simulink model "AFC_FFNN_trainscg_15_15_15_15_15_ctr_Nor_July_15"  (R2021a)
settings: Solver=VariableStepAuto  StartTime=0.0  StopTime=10.0  RelTol=1e-3
libraries: neural x82
(part 2 of 3)

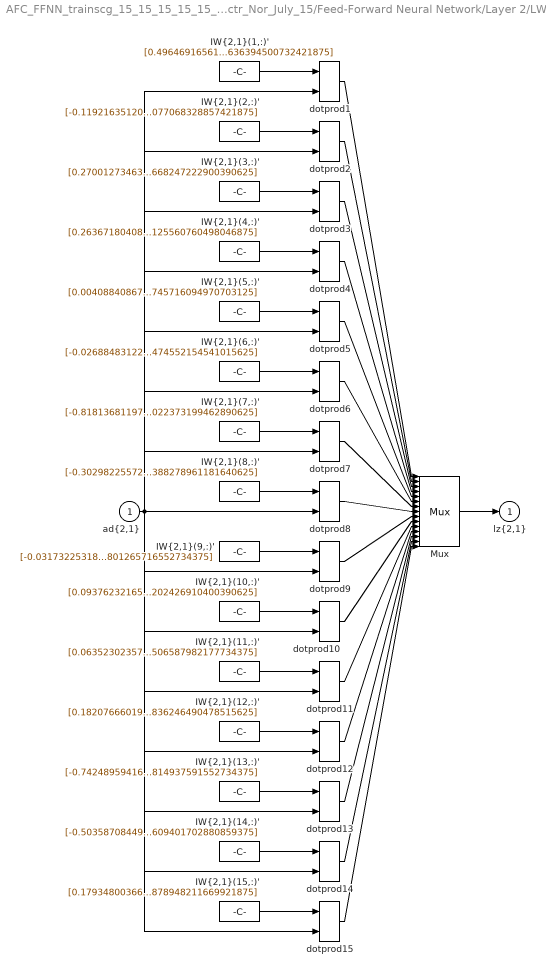
== system AFC_FFNN_trainscg_15_15_15_15_15_ctr_Nor_July_15/Feed-Forward Neural Network/Layer 2/LW{2,1} ==
  "ad{2,1}" : Inport  PortDimensions=15
      mask Display: e = 0.06;c1 = [120 230 180]/255;c2 = ([120 230 180]+0)/(256+128);c3 = ([120 230 180]+128)/(256+128);patch([0 1 1 0],[0 0 1 1],c1);patch([0 1 1 1-e 1-e 0+e],[0 0 1 1-e 0+e 0+e],c2);patch([0 0 1 1-e 0+e 0+e],[0 1 1 1-e 1-e 0+e],c3);plot([0 1 1 0 0],[0 0 1 1 0]);
  "IW{2,1}(1,:)'" : Constant  Value=[0.49646916561011245061507679565693251788616180419921875;0.77996133484927110401940808515064418315887451171875;-0.4843167782638080343105002611991949379444122314453125;0.91967297978227990906674449433921836316585540771484375;0.8707941521523403505256055723293684422969818115234375;0.5037557738819355979131842104834504425525665283203125;-0.7017295301971968601861817660392262041568756103515625;0.309274426520241119131782170370570383965969085693359375;0.90641457105355194290297049519722349941730499267578125;0.10882574325775402901417265866257366724312305450439453125;0.90673057127212108863290040972060523927211761474609375;-0.80524588547048792097626801478327251970767974853515625;0.104579561651616914641493849558173678815364837646484375;-0.386551898471740595919499128285679034888744354248046875;0.4908219201017736121883672240073792636394500732421875]
      mask Display: e = 0.06;c1 = [120 150 230]/255;c2 = ([120 150 230]+0)/383;c3 = ([120 150 230]+128)/383;patch([0 1 1 0],[0 0 1 1],c1);patch([0 1 1 1-e 1-e 0+e],[0 0 1 1-e 0+e 0+e],c2);patch([0 0 1 1-e 0+e 0+e],[0 1 1 1-e 1-e 0+e],c3);plot([0 1 1 0 0],[0 0 1 1 0]);disp('weights');
  "IW{2,1}(10,:)'" : Constant  Value=[0.0937623216569043460566490466590039432048797607421875;0.77106293047639129500936405747779645025730133056640625;0.4586134724193680067827472157659940421581268310546875;-0.7860483088632481685209540955838747322559356689453125;-0.52866293231569916333256742291268892586231231689453125;0.6383602490350686053943718434311449527740478515625;0.342034306689907363629998826581868343055248260498046875;0.212238388955804213598099750015535391867160797119140625;-0.976573937691504578850754114682786166667938232421875;0.64814439757751340920322036254219710826873779296875;-0.88015675771774992686147243148298002779483795166015625;-0.537524641968443628314844318083487451076507568359375;-0.552249744431198674732286235666833817958831787109375;-0.32473785236878993654130454160622321069240570068359375;-0.11032019079443211584390382995479740202426910400390625]
      mask Display: e = 0.06;c1 = [120 150 230]/255;c2 = ([120 150 230]+0)/383;c3 = ([120 150 230]+128)/383;patch([0 1 1 0],[0 0 1 1],c1);patch([0 1 1 1-e 1-e 0+e],[0 0 1 1-e 0+e 0+e],c2);patch([0 0 1 1-e 0+e 0+e],[0 1 1 1-e 1-e 0+e],c3);plot([0 1 1 0 0],[0 0 1 1 0]);disp('weights');
  "IW{2,1}(11,:)'" : Constant  Value=[0.06352302357512840114139862635056488215923309326171875;0.77580634612318088993987430512788705527782440185546875;0.4976683056216459899445681003271602094173431396484375;0.710615284497925880913271612371318042278289794921875;0.0284508200153920677577534803504022420383989810943603515625;-0.4262598504785959363516667508520185947418212890625;0.79535543465944924523824965945095755159854888916015625;-0.50420641521105835636262781918048858642578125;-0.78178862131788517952912798136821947991847991943359375;0.64520731580435242147331109663355164229869842529296875;0.8267663858165315016179874874069355428218841552734375;-0.480465110495678582314127424979233182966709136962890625;0.53645329785536877142959610864636488258838653564453125;0.09182180567506821600165523022951674647629261016845703125;-0.2422337966092920902294594043269171379506587982177734375]
      mask Display: e = 0.06;c1 = [120 150 230]/255;c2 = ([120 150 230]+0)/383;c3 = ([120 150 230]+128)/383;patch([0 1 1 0],[0 0 1 1],c1);patch([0 1 1 1-e 1-e 0+e],[0 0 1 1-e 0+e 0+e],c2);patch([0 0 1 1-e 0+e 0+e],[0 1 1 1-e 1-e 0+e],c3);plot([0 1 1 0 0],[0 0 1 1 0]);disp('weights');
  "IW{2,1}(12,:)'" : Constant  Value=[0.182076660191047789982832227906328625977039337158203125;0.0361498754295182800344576889983727596700191497802734375;0.943422814506380991161904603359289467334747314453125;-0.07051674807384201992821459725746535696089267730712890625;-0.91829558979760783632428911005263216793537139892578125;0.7502905528531134127234736297396011650562286376953125;0.496483911800009891646112691887537948787212371826171875;0.59923945203563711014993486969615332782268524169921875;-0.3292028577878360895425657872692681849002838134765625;-0.13105378107113896390956142568029463291168212890625;0.80434019538809276017587990281754173338413238525390625;0.249007566369504773629017790881334803998470306396484375;-0.89566786392105457448309380197315476834774017333984375;0.9758812474243507839588573915534652769565582275390625;-0.3177526207662977331125375712872482836246490478515625]
      mask Display: e = 0.06;c1 = [120 150 230]/255;c2 = ([120 150 230]+0)/383;c3 = ([120 150 230]+128)/383;patch([0 1 1 0],[0 0 1 1],c1);patch([0 1 1 1-e 1-e 0+e],[0 0 1 1-e 0+e 0+e],c2);patch([0 0 1 1-e 0+e 0+e],[0 1 1 1-e 1-e 0+e],c3);plot([0 1 1 0 0],[0 0 1 1 0]);disp('weights');
  "IW{2,1}(13,:)'" : Constant  Value=[-0.7424895941637081886455007406766526401042938232421875;-0.856648876074442622297056004754267632961273193359375;0.4489983138356112846167889074422419071197509765625;0.0342511534493581404348105934332124888896942138671875;-0.1478990255038865608838705156813375651836395263671875;-0.727415351703474044597896863706409931182861328125;-0.7367400157489829570778283596155233681201934814453125;0.0653226259463746128375305488589219748973846435546875;-0.089870329604618603980270563624799251556396484375;0.0129175888645709502355884978896938264369964599609375;0.8733140785372424108601308034849353134632110595703125;-0.2333190812499730260043406815384514629840850830078125;-0.72095782901882099480417309678159654140472412109375;-0.6008520238705161720105252243229188024997711181640625;-0.9615455944680115774048090315773151814937591552734375]
      mask Display: e = 0.06;c1 = [120 150 230]/255;c2 = ([120 150 230]+0)/383;c3 = ([120 150 230]+128)/383;patch([0 1 1 0],[0 0 1 1],c1);patch([0 1 1 1-e 1-e 0+e],[0 0 1 1-e 0+e 0+e],c2);patch([0 0 1 1-e 0+e 0+e],[0 1 1 1-e 1-e 0+e],c3);plot([0 1 1 0 0],[0 0 1 1 0]);disp('weights');
  "IW{2,1}(14,:)'" : Constant  Value=[-0.50358708449105638038645338383503258228302001953125;0.98956782330111947576511965962708927690982818603515625;-0.2361487675618059167703677303506992757320404052734375;0.007202825434977723484397671427359455265104770660400390625;-0.54195442663654513903992437917622737586498260498046875;0.95067385879104904233827255666255950927734375;-0.492871953524475603369836562706041149795055389404296875;-0.838459952423429744072791436337865889072418212890625;0.7937041538789466610381850841804407536983489990234375;0.59786126522488303169922119195689447224140167236328125;0.40169531108736389324320725791039876639842987060546875;-0.11999535239950331888536538826883770525455474853515625;0.3818939688303688573256522431620396673679351806640625;0.28629620337122674289531687463750131428241729736328125;0.306668631161549354313677895333967171609401702880859375]
      mask Display: e = 0.06;c1 = [120 150 230]/255;c2 = ([120 150 230]+0)/383;c3 = ([120 150 230]+128)/383;patch([0 1 1 0],[0 0 1 1],c1);patch([0 1 1 1-e 1-e 0+e],[0 0 1 1-e 0+e 0+e],c2);patch([0 0 1 1-e 0+e 0+e],[0 1 1 1-e 1-e 0+e],c3);plot([0 1 1 0 0],[0 0 1 1 0]);disp('weights');
  "IW{2,1}(15,:)'" : Constant  Value=[0.1793480036698109625348251938703469932079315185546875;-0.1774866557153116364276002059341408312320709228515625;0.0058018808544819666650482758996076881885528564453125;-0.43136233850821792401575294206850230693817138671875;0.6441880721956698696573084816918708384037017822265625;0.9393437732971190445852016637218184769153594970703125;-0.4988861248860751995692908167256973683834075927734375;0.1004589318309039303045437918626703321933746337890625;-0.874463826702308377747385748079977929592132568359375;0.301052562896285902382942367694340646266937255859375;-0.477452557381994768803679107804782688617706298828125;-0.759402127653759695391499917604960501194000244140625;-0.9407295984391181864481268348754383623600006103515625;-0.7407365473768721120251257161726243793964385986328125;0.8829622103937289079311767636681906878948211669921875]
      mask Display: e = 0.06;c1 = [120 150 230]/255;c2 = ([120 150 230]+0)/383;c3 = ([120 150 230]+128)/383;patch([0 1 1 0],[0 0 1 1],c1);patch([0 1 1 1-e 1-e 0+e],[0 0 1 1-e 0+e 0+e],c2);patch([0 0 1 1-e 0+e 0+e],[0 1 1 1-e 1-e 0+e],c3);plot([0 1 1 0 0],[0 0 1 1 0]);disp('weights');
  "IW{2,1}(2,:)'" : Constant  Value=[-0.11921635120059757839694469794267206452786922454833984375;-0.607546895104995154923699374194256961345672607421875;0.5900632710409168257825740511179901659488677978515625;-0.138270521887720487796968882321380078792572021484375;0.94863459152685891684342323060263879597187042236328125;0.108212254673193175591450199135579168796539306640625;0.6336456199801230315671318749082274734973907470703125;-0.852210835717297499058986431919038295745849609375;0.499621559800357439851126173380180262029170989990234375;0.324437729528092744235578948064357973635196685791015625;-0.450664172986721733860093763723853044211864471435546875;-0.53748757708461780691067133375327102839946746826171875;0.1466756409986354758867577174896723590791225433349609375;0.9207406241604727537009011939517222344875335693359375;0.6230024512652061474682341213338077068328857421875]
      mask Display: e = 0.06;c1 = [120 150 230]/255;c2 = ([120 150 230]+0)/383;c3 = ([120 150 230]+128)/383;patch([0 1 1 0],[0 0 1 1],c1);patch([0 1 1 1-e 1-e 0+e],[0 0 1 1-e 0+e 0+e],c2);patch([0 0 1 1-e 0+e 0+e],[0 1 1 1-e 1-e 0+e],c3);plot([0 1 1 0 0],[0 0 1 1 0]);disp('weights');
  "IW{2,1}(3,:)'" : Constant  Value=[0.2700127346397784844356237954343669116497039794921875;-0.9047528966046705090064961041207425296306610107421875;-0.430330309352361606300974017358385026454925537109375;-0.6030524532782468583036461495794355869293212890625;0.6380385707500888514687176211737096309661865234375;0.54795002035806472662216037861071527004241943359375;0.005250284302730445773477185866795480251312255859375;-0.1241388584709621767387943691574037075042724609375;-0.535917014359012622293221284053288400173187255859375;-0.7535723587361520259264580090530216693878173828125;-0.6954156221470046972399359219707548618316650390625;-0.1377055300142842053645608757506124675273895263671875;0.9674587418212110545567838926217518746852874755859375;-0.366043734123321140572215881547890603542327880859375;0.27252194091142545318007250898517668247222900390625]
      mask Display: e = 0.06;c1 = [120 150 230]/255;c2 = ([120 150 230]+0)/383;c3 = ([120 150 230]+128)/383;patch([0 1 1 0],[0 0 1 1],c1);patch([0 1 1 1-e 1-e 0+e],[0 0 1 1-e 0+e 0+e],c2);patch([0 0 1 1-e 0+e 0+e],[0 1 1 1-e 1-e 0+e],c3);plot([0 1 1 0 0],[0 0 1 1 0]);disp('weights');
  "IW{2,1}(4,:)'" : Constant  Value=[0.263671804087154904028267310422961600124835968017578125;-0.088848657628518290518826461266144178807735443115234375;0.319605914056265039135951155913062393665313720703125;0.43228381383499936418957076966762542724609375;-0.50480747820906402001384094546665437519550323486328125;0.5334080567160881525268223413149826228618621826171875;0.24319585957480349680537301537697203457355499267578125;0.0781634291431403394057042532949708402156829833984375;0.42457360577352798447492432387662120163440704345703125;0.419709979053071668975150032565579749643802642822265625;0.064052803186310125482805233332328498363494873046875;0.1443572233574179353166044847966986708343029022216796875;0.499054679010293267271691775022190995514392852783203125;-0.95638137624631947009135046755545772612094879150390625;0.73648140912501414145907574493321590125560760498046875]
      mask Display: e = 0.06;c1 = [120 150 230]/255;c2 = ([120 150 230]+0)/383;c3 = ([120 150 230]+128)/383;patch([0 1 1 0],[0 0 1 1],c1);patch([0 1 1 1-e 1-e 0+e],[0 0 1 1-e 0+e 0+e],c2);patch([0 0 1 1-e 0+e 0+e],[0 1 1 1-e 1-e 0+e],c3);plot([0 1 1 0 0],[0 0 1 1 0]);disp('weights');
  "IW{2,1}(5,:)'" : Constant  Value=[0.00408840867784126572870295746042756945826113224029541015625;0.09388048935012498208418918466122704558074474334716796875;-0.991924688688980982220755322487093508243560791015625;-0.8552316983080421319840525029576383531093597412109375;-0.1911860906079498878540334771969355642795562744140625;0.366618630720363825048480066470801830291748046875;0.7860653630786631484994586571701802313327789306640625;0.37038892020122304860052508956869132816791534423828125;-0.8905075787511116391925725110922940075397491455078125;-0.50182237106303106966009863754152320325374603271484375;0.7785018803667196340967393553000874817371368408203125;0.7206772319558594208643853562534786760807037353515625;-0.07958944169128155665671187080079107545316219329833984375;0.8513328940182223192323363036848604679107666015625;-0.9719425482959789253101234862697310745716094970703125]
      mask Display: e = 0.06;c1 = [120 150 230]/255;c2 = ([120 150 230]+0)/383;c3 = ([120 150 230]+128)/383;patch([0 1 1 0],[0 0 1 1],c1);patch([0 1 1 1-e 1-e 0+e],[0 0 1 1-e 0+e 0+e],c2);patch([0 0 1 1-e 0+e 0+e],[0 1 1 1-e 1-e 0+e],c3);plot([0 1 1 0 0],[0 0 1 1 0]);disp('weights');
  "IW{2,1}(6,:)'" : Constant  Value=[-0.0268848312263405588018461145338733331300318241119384765625;0.9246644738401335050781426616595126688480377197265625;-0.3050290799498984739557272405363619327545166015625;0.38414616541861434928506469077547080814838409423828125;0.034637294652763044033871864257889683358371257781982421875;0.625021902709288923460917430929839611053466796875;0.5043207504740092605999279840034432709217071533203125;0.1342838675116662938702205565277836285531520843505859375;-0.271313482373797321134389903818373568356037139892578125;0.4706688023118104080566581615130417048931121826171875;0.192185046668555903348618585368967615067958831787109375;0.903737226583765984599949661060236394405364990234375;-0.191130177012016011506290169563726522028446197509765625;-0.45184982043038257604194996019941754639148712158203125;-0.45605259254523444756301842062384821474552154541015625]
      mask Display: e = 0.06;c1 = [120 150 230]/255;c2 = ([120 150 230]+0)/383;c3 = ([120 150 230]+128)/383;patch([0 1 1 0],[0 0 1 1],c1);patch([0 1 1 1-e 1-e 0+e],[0 0 1 1-e 0+e 0+e],c2);patch([0 0 1 1-e 0+e 0+e],[0 1 1 1-e 1-e 0+e],c3);plot([0 1 1 0 0],[0 0 1 1 0]);disp('weights');
  "IW{2,1}(7,:)'" : Constant  Value=[-0.8181368119719962805902468971908092498779296875;-0.2417652257721003561385941793560050427913665771484375;0.77475446764487099216012211400084197521209716796875;-0.8479136503999418206234395256615243852138519287109375;-0.1962586542624291663372559924027882516384124755859375;-0.8289192649386392108823429225594736635684967041015625;-0.5728176091748220510879718858632259070873260498046875;-0.509054777740965302967879324569366872310638427734375;0.595048053803708398845628835260868072509765625;-0.0668896360863564520826685111387632787227630615234375;-0.723707884416889601908451368217356503009796142578125;-0.110236535200048280103146680630743503570556640625;-0.0815360751524158988701174166635610163211822509765625;-0.7837666978321446986655018918099813163280487060546875;0.676385977534560201007707291864790022373199462890625]
      mask Display: e = 0.06;c1 = [120 150 230]/255;c2 = ([120 150 230]+0)/383;c3 = ([120 150 230]+128)/383;patch([0 1 1 0],[0 0 1 1],c1);patch([0 1 1 1-e 1-e 0+e],[0 0 1 1-e 0+e 0+e],c2);patch([0 0 1 1-e 0+e 0+e],[0 1 1 1-e 1-e 0+e],c3);plot([0 1 1 0 0],[0 0 1 1 0]);disp('weights');
  "IW{2,1}(8,:)'" : Constant  Value=[-0.302982255725591453909828487667255103588104248046875;0.8981066832894628593209063183167017996311187744140625;0.7377501160157395876382224741973914206027984619140625;-0.51436050278973510785363032482564449310302734375;-0.974697580153902176647306987433694303035736083984375;0.7051429342498158892027504407451488077640533447265625;0.4605206164095310139572347907233051955699920654296875;-0.373094973925372386247545364312827587127685546875;0.162026455868859553532956851995550096035003662109375;0.0954318321609530784144226345233619213104248046875;-0.53521495323957424261607229709625244140625;-0.0899306950871696653138087640400044620037078857421875;-0.41688631732145697839087006286717951297760009765625;-0.75233462966951680783722622436471283435821533203125;-0.5567396324852271760619260021485388278961181640625]
      mask Display: e = 0.06;c1 = [120 150 230]/255;c2 = ([120 150 230]+0)/383;c3 = ([120 150 230]+128)/383;patch([0 1 1 0],[0 0 1 1],c1);patch([0 1 1 1-e 1-e 0+e],[0 0 1 1-e 0+e 0+e],c2);patch([0 0 1 1-e 0+e 0+e],[0 1 1 1-e 1-e 0+e],c3);plot([0 1 1 0 0],[0 0 1 1 0]);disp('weights');
  "IW{2,1}(9,:)'" : Constant  Value=[-0.03173225318246419845991113106720149517059326171875;-0.552686190513204333996100103831849992275238037109375;0.540447992482629313570896556484512984752655029296875;0.50729806833549417888207244686782360076904296875;-0.1229728520261097468591060533071868121623992919921875;0.612215314341371996675889022299088537693023681640625;-0.6820196650305467844788154252455569803714752197265625;0.7640746318530091674148252423037774860858917236328125;0.9475084056062905712991550899459980428218841552734375;0.406609182665139012868849022197537124156951904296875;-0.231903100212810020508413799689151346683502197265625;-0.83148171255660230372086516581475734710693359375;-0.5010392717716840582653503588517196476459503173828125;-0.443925165630052021015217178501188755035400390625;0.3313515085669587190153606570675037801265716552734375]
      mask Display: e = 0.06;c1 = [120 150 230]/255;c2 = ([120 150 230]+0)/383;c3 = ([120 150 230]+128)/383;patch([0 1 1 0],[0 0 1 1],c1);patch([0 1 1 1-e 1-e 0+e],[0 0 1 1-e 0+e 0+e],c2);patch([0 0 1 1-e 0+e 0+e],[0 1 1 1-e 1-e 0+e],c3);plot([0 1 1 0 0],[0 0 1 1 0]);disp('weights');
  Mux : Mux  Inputs=15
      mask Display: e = 0.06;c1 = [120 150 230]/255;c2 = ([120 150 230]+0)/383;c3 = ([120 150 230]+128)/383;patch([0 1 1 0],[0 0 1 1],c1);patch([0 1 1 1-e 1-e 0+e],[0 0 1 1-e 0+e 0+e],c2);patch([0 0 1 1-e 0+e 0+e],[0 1 1 1-e 1-e 0+e],c3);plot([0 1 1 0 0],[0 0 1 1 0]);disp('Mux');
  dotprod{1..15} (15 alike) : neural/Weight Functions/dotprod
  "lz{2,1}" : Outport
      mask Display: e = 0.06;c1 = [120 230 180]/255;c2 = ([120 230 180]+0)/(256+128);c3 = ([120 230 180]+128)/(256+128);patch([0 1 1 0],[0 0 1 1],c1);patch([0 1 1 1-e 1-e 0+e],[0 0 1 1-e 0+e 0+e],c2);patch([0 0 1 1-e 0+e 0+e],[0 1 1 1-e 1-e 0+e],c3);plot([0 1 1 0 0],[0 0 1 1 0]);
  wires:
  "IW{2,1}(1,:)'"/1 -> dotprod1/1
  "ad{2,1}"/1 -> dotprod1/2, dotprod2/2, dotprod3/2, dotprod4/2, dotprod5/2, dotprod6/2, dotprod7/2, dotprod8/2, dotprod9/2, dotprod10/2, dotprod11/2, dotprod12/2, dotprod13/2, dotprod14/2, dotprod15/2
  dotprod1/1 -> Mux/1
  "IW{2,1}(2,:)'"/1 -> dotprod2/1
  dotprod2/1 -> Mux/2
  "IW{2,1}(3,:)'"/1 -> dotprod3/1
  dotprod3/1 -> Mux/3
  "IW{2,1}(4,:)'"/1 -> dotprod4/1
  dotprod4/1 -> Mux/4
  "IW{2,1}(5,:)'"/1 -> dotprod5/1
  dotprod5/1 -> Mux/5
  "IW{2,1}(6,:)'"/1 -> dotprod6/1
  dotprod6/1 -> Mux/6
  "IW{2,1}(7,:)'"/1 -> dotprod7/1
  dotprod7/1 -> Mux/7
  "IW{2,1}(8,:)'"/1 -> dotprod8/1
  dotprod8/1 -> Mux/8
  "IW{2,1}(9,:)'"/1 -> dotprod9/1
  dotprod9/1 -> Mux/9
  "IW{2,1}(10,:)'"/1 -> dotprod10/1
  dotprod10/1 -> Mux/10
  "IW{2,1}(11,:)'"/1 -> dotprod11/1
  dotprod11/1 -> Mux/11
  "IW{2,1}(12,:)'"/1 -> dotprod12/1
  dotprod12/1 -> Mux/12
  "IW{2,1}(13,:)'"/1 -> dotprod13/1
  dotprod13/1 -> Mux/13
  "IW{2,1}(14,:)'"/1 -> dotprod14/1
  dotprod14/1 -> Mux/14
  "IW{2,1}(15,:)'"/1 -> dotprod15/1
  dotprod15/1 -> Mux/15
  Mux/1 -> "lz{2,1}"/1

== system AFC_FFNN_trainscg_15_15_15_15_15_ctr_Nor_July_15/Feed-Forward Neural Network/Layer 3/Delays 1 ==
  "p{3}" : Inport  PortDimensions=15
      mask Display: e = 0.06;c1 = [120 230 180]/255;c2 = ([120 230 180]+0)/(256+128);c3 = ([120 230 180]+128)/(256+128);patch([0 1 1 0],[0 0 1 1],c1);patch([0 1 1 1-e 1-e 0+e],[0 0 1 1-e 0+e 0+e],c2);patch([0 0 1 1-e 0+e 0+e],[0 1 1 1-e 1-e 0+e],c3);plot([0 1 1 0 0],[0 0 1 1 0]);
  mux : Mux  Inputs=1
      mask Display: e = 0.06;c1 = [120 150 230]/255;c2 = ([120 150 230]+0)/383;c3 = ([120 150 230]+128)/383;patch([0 1 1 0],[0 0 1 1],c1);patch([0 1 1 1-e 1-e 0+e],[0 0 1 1-e 0+e 0+e],c2);patch([0 0 1 1-e 0+e 0+e],[0 1 1 1-e 1-e 0+e],c3);plot([0 1 1 0 0],[0 0 1 1 0]);disp('Mux')
  "pd{3,2}" : Outport
      mask Display: e = 0.06;c1 = [120 230 180]/255;c2 = ([120 230 180]+0)/(256+128);c3 = ([120 230 180]+128)/(256+128);patch([0 1 1 0],[0 0 1 1],c1);patch([0 1 1 1-e 1-e 0+e],[0 0 1 1-e 0+e 0+e],c2);patch([0 0 1 1-e 0+e 0+e],[0 1 1 1-e 1-e 0+e],c3);plot([0 1 1 0 0],[0 0 1 1 0]);
  wires:
  "p{3}"/1 -> mux/1
  mux/1 -> "pd{3,2}"/1

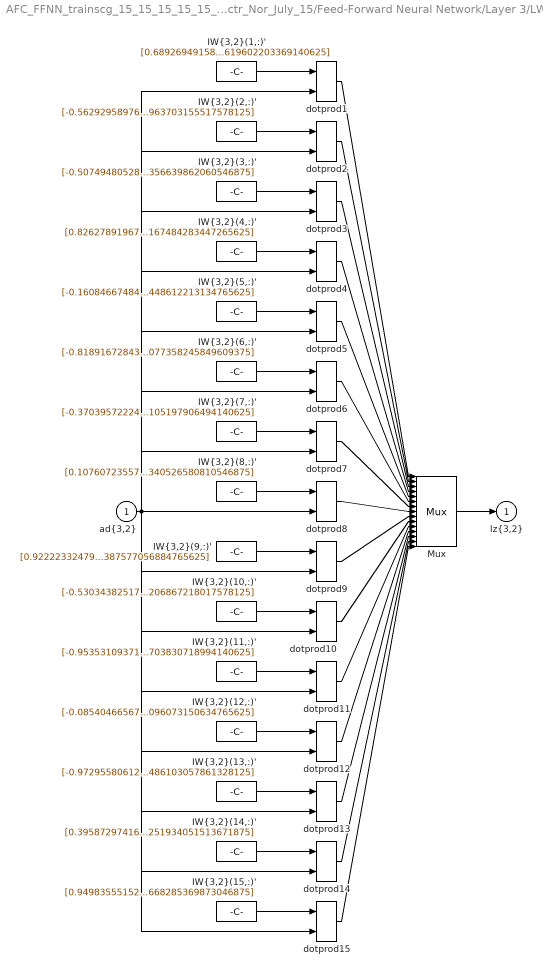
== system AFC_FFNN_trainscg_15_15_15_15_15_ctr_Nor_July_15/Feed-Forward Neural Network/Layer 3/LW{3,2} ==
  "ad{3,2}" : Inport  PortDimensions=15
      mask Display: e = 0.06;c1 = [120 230 180]/255;c2 = ([120 230 180]+0)/(256+128);c3 = ([120 230 180]+128)/(256+128);patch([0 1 1 0],[0 0 1 1],c1);patch([0 1 1 1-e 1-e 0+e],[0 0 1 1-e 0+e 0+e],c2);patch([0 0 1 1-e 0+e 0+e],[0 1 1 1-e 1-e 0+e],c3);plot([0 1 1 0 0],[0 0 1 1 0]);
  "IW{3,2}(1,:)'" : Constant  Value=[0.68926949158478090229351664675050415098667144775390625;-0.64905444834060321834812157248961739242076873779296875;0.7831486761913992733497025255928747355937957763671875;-0.61261901862496159765214542858302593231201171875;0.6429042951633501257191483091446571052074432373046875;-0.414752693122203475173392916985903866589069366455078125;-0.0962218095989033628256947849877178668975830078125;-0.670945891090518831134659194503910839557647705078125;0.60892969517095618670055046095512807369232177734375;0.132741198039494523452930252460646443068981170654296875;-0.057600601034548538914581428116434835828840732574462890625;0.486068283333658868183846379906754009425640106201171875;-0.794885979199396519589981835451908409595489501953125;-0.69121066553226617745764315259293653070926666259765625;-0.7117527019887506245510166991152800619602203369140625]
      mask Display: e = 0.06;c1 = [120 150 230]/255;c2 = ([120 150 230]+0)/383;c3 = ([120 150 230]+128)/383;patch([0 1 1 0],[0 0 1 1],c1);patch([0 1 1 1-e 1-e 0+e],[0 0 1 1-e 0+e 0+e],c2);patch([0 0 1 1-e 0+e 0+e],[0 1 1 1-e 1-e 0+e],c3);plot([0 1 1 0 0],[0 0 1 1 0]);disp('weights');
  "IW{3,2}(10,:)'" : Constant  Value=[-0.53034382517854672389745473992661572992801666259765625;0.86697467324738131111416805651970207691192626953125;0.1227983085759849490870010413345880806446075439453125;0.1020682543837800881902921901200897991657257080078125;0.316351772540197029304209763722610659897327423095703125;-0.282980718830822819409576140969875268638134002685546875;-0.00364319955774927706215748912654817104339599609375;0.0611023243564268181415854996885173022747039794921875;-0.4933274183952125468977101263590157032012939453125;-0.192458458377915475612240925329388119280338287353515625;-0.68593701415923480357861308220890350639820098876953125;-0.262855327129308202760427093380712904036045074462890625;-0.8793423223448504355559407485998235642910003662109375;0.51315921379568474325338911512517370283603668212890625;-0.38244919573806601675869387690909206867218017578125]
      mask Display: e = 0.06;c1 = [120 150 230]/255;c2 = ([120 150 230]+0)/383;c3 = ([120 150 230]+128)/383;patch([0 1 1 0],[0 0 1 1],c1);patch([0 1 1 1-e 1-e 0+e],[0 0 1 1-e 0+e 0+e],c2);patch([0 0 1 1-e 0+e 0+e],[0 1 1 1-e 1-e 0+e],c3);plot([0 1 1 0 0],[0 0 1 1 0]);disp('weights');
  "IW{3,2}(11,:)'" : Constant  Value=[-0.95353109371107824809854491832084022462368011474609375;-0.0106801252669140971096606307355614262633025646209716796875;-0.13341806801815270233646515407599508762359619140625;0.9189527235657564130377750188927166163921356201171875;-0.71682661094343114172033892828039824962615966796875;-0.444461641217060776654079745640046894550323486328125;0.212257352710709223941876189201138913631439208984375;-0.9327321645290667095906655958970077335834503173828125;-0.05127212985187412641607807017862796783447265625;-0.7195320830771059217312313194270245730876922607421875;0.95557244312461409041503657135763205587863922119140625;-0.84607443827369011035699486455996520817279815673828125;0.5912676567652963566246171467355452477931976318359375;-0.4259251297044659434476443493622355163097381591796875;0.1932521141071052994675483205355703830718994140625]
      mask Display: e = 0.06;c1 = [120 150 230]/255;c2 = ([120 150 230]+0)/383;c3 = ([120 150 230]+128)/383;patch([0 1 1 0],[0 0 1 1],c1);patch([0 1 1 1-e 1-e 0+e],[0 0 1 1-e 0+e 0+e],c2);patch([0 0 1 1-e 0+e 0+e],[0 1 1 1-e 1-e 0+e],c3);plot([0 1 1 0 0],[0 0 1 1 0]);disp('weights');
  "IW{3,2}(12,:)'" : Constant  Value=[-0.0854046656743794319055496089276857674121856689453125;-0.0516975049611743120436813114793039858341217041015625;0.6786291324143771674926028936170041561126708984375;0.99883997819401049156340377521701157093048095703125;-0.9424632651980908715216855853213928639888763427734375;-0.1453470674596208933593288747943006455898284912109375;-0.7388862796930426579677941845147870481014251708984375;0.981669669379983123036481629242189228534698486328125;0.8675045904703189147966213567997328937053680419921875;0.0739123875832008447872567558079026639461517333984375;-0.5176211250662430263247415496152825653553009033203125;-0.9231613363171853325894744557444937527179718017578125;0.1173255985049836969125180985429324209690093994140625;-0.9587271311368128490215667625307105481624603271484375;-0.7137937826656772788425087128416635096073150634765625]
      mask Display: e = 0.06;c1 = [120 150 230]/255;c2 = ([120 150 230]+0)/383;c3 = ([120 150 230]+128)/383;patch([0 1 1 0],[0 0 1 1],c1);patch([0 1 1 1-e 1-e 0+e],[0 0 1 1-e 0+e 0+e],c2);patch([0 0 1 1-e 0+e 0+e],[0 1 1 1-e 1-e 0+e],c3);plot([0 1 1 0 0],[0 0 1 1 0]);disp('weights');
  "IW{3,2}(13,:)'" : Constant  Value=[-0.9729558061272209901204632842564024031162261962890625;0.148019201281444134910003640470677055418491363525390625;-0.9601201263948049291485631329123862087726593017578125;-0.457150030592506084747839167903293855488300323486328125;0.881381558568999690095324694993905723094940185546875;-0.578115263594495498722380943945609033107757568359375;-0.5573231148004509361015834656427614390850067138671875;-0.4634683435141138119206516421400010585784912109375;-0.0261862264098524644140297823469154536724090576171875;-0.98366029135030164098907334846444427967071533203125;0.9100587127389923036702157332911156117916107177734375;-0.60658409367462218231281667613075114786624908447265625;0.5397436102716650641042406277847476303577423095703125;-0.70489583483044404577100294773117639124393463134765625;0.3715703476170262309352665397454984486103057861328125]
      mask Display: e = 0.06;c1 = [120 150 230]/255;c2 = ([120 150 230]+0)/383;c3 = ([120 150 230]+128)/383;patch([0 1 1 0],[0 0 1 1],c1);patch([0 1 1 1-e 1-e 0+e],[0 0 1 1-e 0+e 0+e],c2);patch([0 0 1 1-e 0+e 0+e],[0 1 1 1-e 1-e 0+e],c3);plot([0 1 1 0 0],[0 0 1 1 0]);disp('weights');
  "IW{3,2}(14,:)'" : Constant  Value=[0.395872974169953817380473992670886218547821044921875;-0.98742185604539167709248204118921421468257904052734375;0.5005797930699971143297943854122422635555267333984375;0.64459120988025608856020198800251819193363189697265625;0.356616175530686307926231393139460124075412750244140625;0.494785064932234119883247558391303755342960357666015625;-0.7257076431667683902304588627885095775127410888671875;0.7573612430550138441276430967263877391815185546875;0.3588984204049230353206212384975515305995941162109375;0.78325236876618908876679370223428122699260711669921875;0.95428037897558570801237465275335125625133514404296875;-0.10244648072712657371763356195515370927751064300537109375;-0.75263446557823865390446371748112142086029052734375;0.663464732529429834784195918473415076732635498046875;-0.9551689522931325893040366281638853251934051513671875]
      mask Display: e = 0.06;c1 = [120 150 230]/255;c2 = ([120 150 230]+0)/383;c3 = ([120 150 230]+128)/383;patch([0 1 1 0],[0 0 1 1],c1);patch([0 1 1 1-e 1-e 0+e],[0 0 1 1-e 0+e 0+e],c2);patch([0 0 1 1-e 0+e 0+e],[0 1 1 1-e 1-e 0+e],c3);plot([0 1 1 0 0],[0 0 1 1 0]);disp('weights');
  "IW{3,2}(15,:)'" : Constant  Value=[0.9498355515277545624286403835867531597614288330078125;-0.1717845436227796174222248737351037561893463134765625;-0.0778938048783024417076603640452958643436431884765625;0.7986556359639991331533792617847211658954620361328125;-0.21212020938234577016601178911514580249786376953125;-0.951507249067342630866050967597402632236480712890625;-0.266562281207658458015430369414389133453369140625;0.1347170460220714627297411425388418138027191162109375;-0.8966633298562920462160263923578895628452301025390625;0.72298581510557990981169496080838143825531005859375;-0.4486463814792076565396428122767247259616851806640625;-0.4543897029028460821109547396190464496612548828125;0.75523401470857454143015274894423782825469970703125;0.3762590257581537311892816433100961148738861083984375;-0.4430234290704671007432580154272727668285369873046875]
      mask Display: e = 0.06;c1 = [120 150 230]/255;c2 = ([120 150 230]+0)/383;c3 = ([120 150 230]+128)/383;patch([0 1 1 0],[0 0 1 1],c1);patch([0 1 1 1-e 1-e 0+e],[0 0 1 1-e 0+e 0+e],c2);patch([0 0 1 1-e 0+e 0+e],[0 1 1 1-e 1-e 0+e],c3);plot([0 1 1 0 0],[0 0 1 1 0]);disp('weights');
  "IW{3,2}(2,:)'" : Constant  Value=[-0.562929589768697002938324658316560089588165283203125;0.165651753034273152564992415136657655239105224609375;0.9568583771587524378077205255976878106594085693359375;0.5560316320103704246236020480864681303501129150390625;-0.238504282118257027178742646356113255023956298828125;0.8005401741912212543184068636037409305572509765625;-0.93901775570367806977856162120588123798370361328125;-0.688989783220818718945110958884470164775848388671875;-0.9128197821751562468506335790152661502361297607421875;-0.763621831076356283318773421342484652996063232421875;-0.935670688003623407524855792871676385402679443359375;-0.68908866271854751772707459167577326297760009765625;-0.269619161332864454294622191810049116611480712890625;0.9672060355241896001388113290886394679546356201171875;-0.0859138894842665923334834587876684963703155517578125]
      mask Display: e = 0.06;c1 = [120 150 230]/255;c2 = ([120 150 230]+0)/383;c3 = ([120 150 230]+128)/383;patch([0 1 1 0],[0 0 1 1],c1);patch([0 1 1 1-e 1-e 0+e],[0 0 1 1-e 0+e 0+e],c2);patch([0 0 1 1-e 0+e 0+e],[0 1 1 1-e 1-e 0+e],c3);plot([0 1 1 0 0],[0 0 1 1 0]);disp('weights');
  "IW{3,2}(3,:)'" : Constant  Value=[-0.5074948052874506121412423453875817358493804931640625;0.77053787988654953711176176511798985302448272705078125;-0.7363382298223342115051082146237604320049285888671875;0.78742202814315975789583035293617285788059234619140625;0.52418306688785365476945798945962451398372650146484375;0.0303079115437369962793301425563186057843267917633056640625;-0.68992151593302697420995173160918056964874267578125;-0.2673862720881918786375308627611957490444183349609375;0.1387208230034355782578359139733947813510894775390625;-0.0227437019702670210896666702637958223931491374969482421875;-0.7903579986247384336905952295637689530849456787109375;-0.71092558778322756385392722222604788839817047119140625;-0.85751150675600040784729571896605193614959716796875;0.66081167614687874589662897051312029361724853515625;-0.4849577362305506067485794119420461356639862060546875]
      mask Display: e = 0.06;c1 = [120 150 230]/255;c2 = ([120 150 230]+0)/383;c3 = ([120 150 230]+128)/383;patch([0 1 1 0],[0 0 1 1],c1);patch([0 1 1 1-e 1-e 0+e],[0 0 1 1-e 0+e 0+e],c2);patch([0 0 1 1-e 0+e 0+e],[0 1 1 1-e 1-e 0+e],c3);plot([0 1 1 0 0],[0 0 1 1 0]);disp('weights');
  "IW{3,2}(4,:)'" : Constant  Value=[0.8262789196706921135415768731036223471164703369140625;0.7796907145922069570787016346002928912639617919921875;0.863358666186659906571776446071453392505645751953125;0.2554357997803824442684117457247339189052581787109375;0.77856833338737863048351073302910663187503814697265625;0.349985156215272985580355680212960578501224517822265625;0.8537423607916221346414431536686606705188751220703125;-0.131939451533888973955299661611206829547882080078125;0.169808359894214166985193514847196638584136962890625;0.2302788227858534597647377495377440936863422393798828125;-0.87119703430520767373224089169525541365146636962890625;0.5464001123132897763667870094650425016880035400390625;0.07753581185590530111539919744245707988739013671875;0.5963829717247104422739312212797813117504119873046875;-0.2857582500055375618330799625255167484283447265625]
      mask Display: e = 0.06;c1 = [120 150 230]/255;c2 = ([120 150 230]+0)/383;c3 = ([120 150 230]+128)/383;patch([0 1 1 0],[0 0 1 1],c1);patch([0 1 1 1-e 1-e 0+e],[0 0 1 1-e 0+e 0+e],c2);patch([0 0 1 1-e 0+e 0+e],[0 1 1 1-e 1-e 0+e],c3);plot([0 1 1 0 0],[0 0 1 1 0]);disp('weights');
  "IW{3,2}(5,:)'" : Constant  Value=[-0.160846674847559878429592572501860558986663818359375;0.5725155963220462940199695367482490837574005126953125;-0.983765381681773742883478917065076529979705810546875;0.9883897465709858831672818268998526036739349365234375;-0.046437458085572487498371430092447553761303424835205078125;-0.8774053710440583575547179862041957676410675048828125;0.3322310252958544651846750639379024505615234375;-0.4657403300045681593388735564076341688632965087890625;0.123325125465898910448458991595543920993804931640625;0.732605515826929565292857660097070038318634033203125;-0.09622216208059765352178516195635893382132053375244140625;-0.90586018869653706087063937957282178103923797607421875;-0.92720323014644545622786608873866498470306396484375;-0.02650061922837831929200547165237367153167724609375;-0.0226346575634099878016058937646448612213134765625]
      mask Display: e = 0.06;c1 = [120 150 230]/255;c2 = ([120 150 230]+0)/383;c3 = ([120 150 230]+128)/383;patch([0 1 1 0],[0 0 1 1],c1);patch([0 1 1 1-e 1-e 0+e],[0 0 1 1-e 0+e 0+e],c2);patch([0 0 1 1-e 0+e 0+e],[0 1 1 1-e 1-e 0+e],c3);plot([0 1 1 0 0],[0 0 1 1 0]);disp('weights');
  "IW{3,2}(6,:)'" : Constant  Value=[-0.8189167284368645827186128371977247297763824462890625;0.061807328063784527927282397286035120487213134765625;0.017844064952306393223580016638152301311492919921875;-0.9692901124822135283665147653664462268352508544921875;-0.0650675268659763883505320336553268134593963623046875;-0.66108982877411648360066465102136135101318359375;0.6150896999685613319996946302126161754131317138671875;-0.9475317479734639558586195562384091317653656005859375;0.27864289333406677684479291201569139957427978515625;-0.0999710377048177445402643570560030639171600341796875;0.255282171335795116107192370691336691379547119140625;0.02957999373653930064165251678787171840667724609375;0.883203184300609844825658001354895532131195068359375;-0.948810814237413868710291353636421263217926025390625;-0.3728712112794771993407039190060459077358245849609375]
      mask Display: e = 0.06;c1 = [120 150 230]/255;c2 = ([120 150 230]+0)/383;c3 = ([120 150 230]+128)/383;patch([0 1 1 0],[0 0 1 1],c1);patch([0 1 1 1-e 1-e 0+e],[0 0 1 1-e 0+e 0+e],c2);patch([0 0 1 1-e 0+e 0+e],[0 1 1 1-e 1-e 0+e],c3);plot([0 1 1 0 0],[0 0 1 1 0]);disp('weights');
  "IW{3,2}(7,:)'" : Constant  Value=[-0.370395722246221359430506936405436135828495025634765625;0.044590764100431772021249088311378727667033672332763671875;0.8785175341474076304848495055921375751495361328125;-0.976943983770184321002716387738473713397979736328125;0.43236263507675920525485935286269523203372955322265625;-0.296324961438232670207781893623177893459796905517578125;-0.789793825881249578202414340921677649021148681640625;0.5878218515385345011026174688595347106456756591796875;0.2276506223106313786530563447740860283374786376953125;-0.28010679864059684351929035983630456030368804931640625;-0.5399230455464418820810124088893644511699676513671875;0.6545030236788258459768030661507509648799896240234375;0.65644071566094197578422608785331249237060546875;0.322146894332130229177124647321761585772037506103515625;0.8296626813005973932746428545215167105197906494140625]
      mask Display: e = 0.06;c1 = [120 150 230]/255;c2 = ([120 150 230]+0)/383;c3 = ([120 150 230]+128)/383;patch([0 1 1 0],[0 0 1 1],c1);patch([0 1 1 1-e 1-e 0+e],[0 0 1 1-e 0+e 0+e],c2);patch([0 0 1 1-e 0+e 0+e],[0 1 1 1-e 1-e 0+e],c3);plot([0 1 1 0 0],[0 0 1 1 0]);disp('weights');
  "IW{3,2}(8,:)'" : Constant  Value=[0.1076072355737454355750770673694205470383167266845703125;0.431186084387213564017571343356394208967685699462890625;0.9569188082777533299605465799686498939990997314453125;0.357552931921336913934084122956846840679645538330078125;-0.335665225712111381373148333295830525457859039306640625;0.301799808964890281526294302238966338336467742919921875;0.032457440638200996119167029974050819873809814453125;-0.86921450426542801181994946091435849666595458984375;0.6065302952189728369347676562028937041759490966796875;0.33424202847897721557757222399231977760791778564453125;-0.09915225011524893272696346002703648991882801055908203125;0.59735452974551439542238995272782631218433380126953125;-0.9641615996222643314439437745022587478160858154296875;0.34897273551590035634006881082314066588878631591796875;-0.4773999403397606311472145534935407340526580810546875]
      mask Display: e = 0.06;c1 = [120 150 230]/255;c2 = ([120 150 230]+0)/383;c3 = ([120 150 230]+128)/383;patch([0 1 1 0],[0 0 1 1],c1);patch([0 1 1 1-e 1-e 0+e],[0 0 1 1-e 0+e 0+e],c2);patch([0 0 1 1-e 0+e 0+e],[0 1 1 1-e 1-e 0+e],c3);plot([0 1 1 0 0],[0 0 1 1 0]);disp('weights');
  "IW{3,2}(9,:)'" : Constant  Value=[0.9222233247908968589712230823352001607418060302734375;-0.9651347018682070455497523653320968151092529296875;0.3126439464082562125213371473364531993865966796875;0.05283618341942375451480984338559210300445556640625;-0.278834754216143121396953574731014668941497802734375;-0.64437479507781869614291281322948634624481201171875;-0.975672238166819472127144763362593948841094970703125;0.1307382086248607411249622600735165178775787353515625;-0.1294502888130011353240433891187421977519989013671875;-0.634352160035149825745293128420598804950714111328125;-0.8981519511431492741593274331535212695598602294921875;-0.318787575353978613890149063081480562686920166015625;-0.4154144334619822576115666379337199032306671142578125;-0.465902387041180698901143841794691979885101318359375;-0.3111476799713577268136077691451646387577056884765625]
      mask Display: e = 0.06;c1 = [120 150 230]/255;c2 = ([120 150 230]+0)/383;c3 = ([120 150 230]+128)/383;patch([0 1 1 0],[0 0 1 1],c1);patch([0 1 1 1-e 1-e 0+e],[0 0 1 1-e 0+e 0+e],c2);patch([0 0 1 1-e 0+e 0+e],[0 1 1 1-e 1-e 0+e],c3);plot([0 1 1 0 0],[0 0 1 1 0]);disp('weights');
  Mux : Mux  Inputs=15
      mask Display: e = 0.06;c1 = [120 150 230]/255;c2 = ([120 150 230]+0)/383;c3 = ([120 150 230]+128)/383;patch([0 1 1 0],[0 0 1 1],c1);patch([0 1 1 1-e 1-e 0+e],[0 0 1 1-e 0+e 0+e],c2);patch([0 0 1 1-e 0+e 0+e],[0 1 1 1-e 1-e 0+e],c3);plot([0 1 1 0 0],[0 0 1 1 0]);disp('Mux');
  dotprod{1..15} (15 alike) : neural/Weight Functions/dotprod
  "lz{3,2}" : Outport
      mask Display: e = 0.06;c1 = [120 230 180]/255;c2 = ([120 230 180]+0)/(256+128);c3 = ([120 230 180]+128)/(256+128);patch([0 1 1 0],[0 0 1 1],c1);patch([0 1 1 1-e 1-e 0+e],[0 0 1 1-e 0+e 0+e],c2);patch([0 0 1 1-e 0+e 0+e],[0 1 1 1-e 1-e 0+e],c3);plot([0 1 1 0 0],[0 0 1 1 0]);
  wires:
  "IW{3,2}(1,:)'"/1 -> dotprod1/1
  "ad{3,2}"/1 -> dotprod1/2, dotprod2/2, dotprod3/2, dotprod4/2, dotprod5/2, dotprod6/2, dotprod7/2, dotprod8/2, dotprod9/2, dotprod10/2, dotprod11/2, dotprod12/2, dotprod13/2, dotprod14/2, dotprod15/2
  dotprod1/1 -> Mux/1
  "IW{3,2}(2,:)'"/1 -> dotprod2/1
  dotprod2/1 -> Mux/2
  "IW{3,2}(3,:)'"/1 -> dotprod3/1
  dotprod3/1 -> Mux/3
  "IW{3,2}(4,:)'"/1 -> dotprod4/1
  dotprod4/1 -> Mux/4
  "IW{3,2}(5,:)'"/1 -> dotprod5/1
  dotprod5/1 -> Mux/5
  "IW{3,2}(6,:)'"/1 -> dotprod6/1
  dotprod6/1 -> Mux/6
  "IW{3,2}(7,:)'"/1 -> dotprod7/1
  dotprod7/1 -> Mux/7
  "IW{3,2}(8,:)'"/1 -> dotprod8/1
  dotprod8/1 -> Mux/8
  "IW{3,2}(9,:)'"/1 -> dotprod9/1
  dotprod9/1 -> Mux/9
  "IW{3,2}(10,:)'"/1 -> dotprod10/1
  dotprod10/1 -> Mux/10
  "IW{3,2}(11,:)'"/1 -> dotprod11/1
  dotprod11/1 -> Mux/11
  "IW{3,2}(12,:)'"/1 -> dotprod12/1
  dotprod12/1 -> Mux/12
  "IW{3,2}(13,:)'"/1 -> dotprod13/1
  dotprod13/1 -> Mux/13
  "IW{3,2}(14,:)'"/1 -> dotprod14/1
  dotprod14/1 -> Mux/14
  "IW{3,2}(15,:)'"/1 -> dotprod15/1
  dotprod15/1 -> Mux/15
  Mux/1 -> "lz{3,2}"/1

== system AFC_FFNN_trainscg_15_15_15_15_15_ctr_Nor_July_15/Feed-Forward Neural Network/Layer 4/Delays 1 ==
  "p{4}" : Inport  PortDimensions=15
      mask Display: e = 0.06;c1 = [120 230 180]/255;c2 = ([120 230 180]+0)/(256+128);c3 = ([120 230 180]+128)/(256+128);patch([0 1 1 0],[0 0 1 1],c1);patch([0 1 1 1-e 1-e 0+e],[0 0 1 1-e 0+e 0+e],c2);patch([0 0 1 1-e 0+e 0+e],[0 1 1 1-e 1-e 0+e],c3);plot([0 1 1 0 0],[0 0 1 1 0]);
  mux : Mux  Inputs=1
      mask Display: e = 0.06;c1 = [120 150 230]/255;c2 = ([120 150 230]+0)/383;c3 = ([120 150 230]+128)/383;patch([0 1 1 0],[0 0 1 1],c1);patch([0 1 1 1-e 1-e 0+e],[0 0 1 1-e 0+e 0+e],c2);patch([0 0 1 1-e 0+e 0+e],[0 1 1 1-e 1-e 0+e],c3);plot([0 1 1 0 0],[0 0 1 1 0]);disp('Mux')
  "pd{4,3}" : Outport
      mask Display: e = 0.06;c1 = [120 230 180]/255;c2 = ([120 230 180]+0)/(256+128);c3 = ([120 230 180]+128)/(256+128);patch([0 1 1 0],[0 0 1 1],c1);patch([0 1 1 1-e 1-e 0+e],[0 0 1 1-e 0+e 0+e],c2);patch([0 0 1 1-e 0+e 0+e],[0 1 1 1-e 1-e 0+e],c3);plot([0 1 1 0 0],[0 0 1 1 0]);
  wires:
  "p{4}"/1 -> mux/1
  mux/1 -> "pd{4,3}"/1
